simulink library "sm_wheel_loader_lib"  (R2025a)
settings: Solver=VariableStepAuto  StartTime=0.0  StopTime=10.0  RelTol=1e-3
undefined symbols (not defined in the file): AToTOrificeVector, BiPOrificeVector, boomHEArea, boomREArea, BToTOrificeVector, fluids, GRake, GToothL, GToothR, HMPST, HydFcnParams, logLoad, Position, PToAOrificeVector, PToBOrificeVector, RakeL, RakeR, testInput, Wheel_Loader, X, Y, Z
libraries: sm_lib x694, fl_lib x183, nesl_utility x74, SimscapeFluids_lib x62, sdl_lib x25, cvt_components_lib x25, simulink_extras x5, $bdroot x4, wheel_loader_contact_lib x4, ee_lib x2, SignalEditorBlockLib x1, batteryecm_lib x1
(part 10 of 26)

== system sm_wheel_loader_lib/Wheel Loader Vehicle/Actuators/Hydraulic/Actuator Steer ==
  Actuator Steer : SimscapeFluids_lib/Isothermal Liquid/Actuators/Double-Acting Actuator (IL)  single_fluid=true  mech_orientation=foundation.enum.MechOrientationTranslational.Positive  piston_area_A=HydFcnParams.steerActuator.headEndArea mm^2  piston_area_B=HydFcnParams.steerActuator.rodEndArea mm^2  stroke=HydFcnParams.steerActuator.stroke mm  dead_volume_A=1e-4 m^3  dead_volume_B=1e-4 m^3  pressure_spec=foundation.enum.pressure_spec.atmospheric  environment_pressure=0.101325 MPa  hardstop_model=simscape.enum.hardstop.smooth  stiff_coeff=1e8 N/m  damping_coeff=1e5 N/(m/s)  transition=0.1 mm  coeff_rest=0.7  v_tol=0.001 m/s  f_tol=0.001 N  cushion_A_spec=simscape.enum.onoff.off  area_plunger_A=boomHEArea/4 mm^2  length_plunger_A=5 mm  area_cushion_orifice_A=5 mm^2  area_leak_plunger_A=1e-7 m^2  p_crack_differential_A=0.01 MPa  press_max_differential_A=0.1 MPa  check_valve_area_max_A=1e-4 m^2  check_valve_area_leak_A=1e-10 m^2  smoothing_factor_A=0  cushion_B_spec=simscape.enum.onoff.off  area_plunger_B=boomREArea/4 mm^2  length_plunger_B=5 mm  area_cushion_orifice_B=5 mm^2  area_leak_plunger_B=1e-7 m^2  p_crack_differential_B=0.01 MPa  press_max_differential_B=0.1 MPa  check_valve_area_max_B=1e-4 m^2  check_valve_area_leak_B=1e-10 m^2  smoothing_factor_B=0  friction_spec=simscape.enum.onoff.on  breakaway_Coulomb_ratio=HydFcnParams.steerActuator.brkawyToCoulRatio  breakaway_velocity=HydFcnParams.steerActuator.brkawyVel m/s  preload_force=HydFcnParams.steerActuator.preloadForce N  Coulomb_coeff=HydFcnParams.steerActuator.coulForceCoef N/Pa  viscous_coeff=HydFcnParams.steerActuator.viscCoeff lbf/(in/s)  leakage_spec=simscape.enum.onoff.off  clearance=1e-4 m  piston_length=0.01 m  displacement_spec=foundation.enum.DisplacementSpec.Calculate  x0=testInput.Active.Steer.p(1)*1000 mm  dynamic_compressibility=simscape.enum.onoff.on  p0_A=HydFcnParams.steerActuator.initHEPr bar  p0_B=HydFcnParams.steerActuator.initREPr bar  p_nominal_A=0.101325 MPa  p_nominal_B=0.101325 MPa
      settings: InternalSimscapePortConfiguration="{\"Bottom\":[],\"Left\":[{\"id\":\"C\",\"label\":\"C\",\"type\":\"foundation.mechanical.translational.translational\"},{\"id\":\"A\",\"label\":\"A\",\"type\":\"foundation.isothermal_liquid.isothermal_liquid\"}],\"Right\":[{\"id\":\"p_out\",\"label\":\"p\",\"type\":\"output\"},{\"id\":\"R\",\"label\":\"R\",\"type\":\"foundation.mechanical.translational.translational\"},{\"id\":\"B\",\"label\":\"B\",\"type\":\"foundation.isothermal_liquid.isothermal_liquid\"}],\"Top\":[]}"
  MTRef : fl_lib/Mechanical/Translational Elements/Mechanical Translational Reference
  PS Terminator : fl_lib/Physical Signals/Sinks/PS Terminator
  A : PMIOPort  Side=Left
  B : PMIOPort  Port=2  Side=Left
  R : PMIOPort  Port=3  Side=Right
  connections:
  Actuator Steer/LConn1 -- MTRef/LConn1
  A/RConn1 -- Actuator Steer/LConn2
  B/RConn1 -- Actuator Steer/RConn3
  R/RConn1 -- Actuator Steer/RConn2
  Actuator Steer/RConn1 -- PS Terminator/LConn1

== system sm_wheel_loader_lib/Wheel Loader Vehicle/Actuators/Hydraulic/Controller ==
  note: Inputs - Outputs:
      |
      | Joystick position for lift (-1 to 1) velocity control - lift arm spool position
      | Joystick position for tilt (-1 to 1) velocity control - tilt spool position
  BusElementIn : Inport  PortName=Cmd  Element=LiftCmd
  BusElementIn1 : Inport  PortName=Cmd  Element=TiltCmd
  Gain : Gain  Gain=5
  Gain1 : Gain  Gain=5
  LiftSpoolPosCmdRateLimit : RateLimiter  RisingSlewLimit=HydFcnParams.liftActCtrl.posSpoolCmdRateLimit  FallingSlewLimit=HydFcnParams.liftActCtrl.negSpoolCmdRateLimit  SampleTimeMode=inherited
  LiftSpoolPosCmdSaturation : Saturate  UpperLimit=HydFcnParams.liftActCtrl.maxSpoolCmd  LowerLimit=HydFcnParams.liftActCtrl.minSpoolCmd
  TiltSpoolPosCmdRateLimit : RateLimiter  RisingSlewLimit=HydFcnParams.tiltActCtrl.posSpoolCmdRateLimit  FallingSlewLimit=HydFcnParams.tiltActCtrl.negSpoolCmdRateLimit  SampleTimeMode=inherited
  TiltSpoolPosCmdSaturation : Saturate  UpperLimit=HydFcnParams.tiltActCtrl.maxSpoolCmd  LowerLimit=HydFcnParams.tiltActCtrl.minSpoolCmd
  Out Bus Element : Outport  PortName=pSpool  Element=tilt
  Out Bus Element1 : Outport  PortName=pSpool  Element=lift
  wires:
  Gain/1 -> LiftSpoolPosCmdSaturation/1
  Gain1/1 -> TiltSpoolPosCmdSaturation/1
  LiftSpoolPosCmdSaturation/1 -> LiftSpoolPosCmdRateLimit/1
  TiltSpoolPosCmdSaturation/1 -> TiltSpoolPosCmdRateLimit/1
  LiftSpoolPosCmdRateLimit/1 -> Out Bus Element1/1  "LiftSpoolPosCmd"
  TiltSpoolPosCmdRateLimit/1 -> Out Bus Element/1  "TiltSpoolCmd"
  BusElementIn1/1 -> Gain1/1
  BusElementIn/1 -> Gain/1

== system sm_wheel_loader_lib/Wheel Loader Vehicle/Actuators/Hydraulic/Implement ==
  A : Inport
  Bucket : Subsystem  VariantControl=Bucket
      mask Display: image('sm_wheel_loader_actuator_bucket_IMAGE.png')
  Grapple : Subsystem  VariantControl=Grapple
      mask Display: image('sm_wheel_loader_actuator_grapple_IMAGE.png')
  Impl : PMIOPort  Side=Right

== system sm_wheel_loader_lib/Wheel Loader Vehicle/Actuators/Hydraulic/Valve Steer ==
  CV SteerA : SimscapeFluids_lib/Isothermal Liquid/Valves & Orifices/Directional Control Valves/Check Valve (IL)  opening_spec=2*(fluids.isothermal_liquid.valves_orifices.enum.opening_spec.linear)-1  pressure_control_spec=fluids.isothermal_liquid.valves_orifices.enum.pressure_control_spec.dp  p_crack_differential=HydFcnParams.checkValves.crackingPrDiff bar  p_crack_gauge=0.1 MPa  press_max_differential=HydFcnParams.checkValves.maxOpeningPrDiff bar  press_max_gauge=0.2 MPa  area_max=HydFcnParams.checkValves.maxOpeningArea mm^2  area_leak="HydFcnParams.checkValves.leakageArea  mm^2"  p_diff_TLU=[0.01 : 0.01 : 0.1] MPa  valve_area_TLU=[1e-10, 1e-05, 2e-05, 3e-05, 4e-05, 5e-05, 6e-05, 7.5e-05, 8.5e-05, .0001] m^2  vol_flow_TLU=[.000358, .045, .11, .191, .284, .39, .505, .63, .764, .905] .* 1e-3 m^3/s  area=inf m^2  Cd=HydFcnParams.checkValves.dischargeCoef  Re_c=HydFcnParams.checkValves.critReynoldsNmbr  smoothing_factor=HydFcnParams.checkValves.smoothingFactor  pressure_recovery=simscape.enum.onoff.off  opening_dynamics=simscape.enum.onoff.off  tau=0.1 s
      settings: InternalSimscapePortConfiguration="{\"Bottom\":[],\"Left\":[{\"id\":\"A\",\"label\":\"A\",\"type\":\"foundation.isothermal_liquid.isothermal_liquid\"}],\"Right\":[{\"id\":\"B\",\"label\":\"B\",\"type\":\"foundation.isothermal_liquid.isothermal_liquid\"}],\"Top\":[]}"
  CV SteerB : SimscapeFluids_lib/Isothermal Liquid/Valves & Orifices/Directional Control Valves/Check Valve (IL)  opening_spec=2*(fluids.isothermal_liquid.valves_orifices.enum.opening_spec.linear)-1  pressure_control_spec=fluids.isothermal_liquid.valves_orifices.enum.pressure_control_spec.dp  p_crack_differential=HydFcnParams.checkValves.crackingPrDiff bar  p_crack_gauge=0.1 MPa  press_max_differential=HydFcnParams.checkValves.maxOpeningPrDiff bar  press_max_gauge=0.2 MPa  area_max=HydFcnParams.checkValves.maxOpeningArea mm^2  area_leak="HydFcnParams.checkValves.leakageArea  mm^2"  p_diff_TLU=[0.01 : 0.01 : 0.1] MPa  valve_area_TLU=[1e-10, 1e-05, 2e-05, 3e-05, 4e-05, 5e-05, 6e-05, 7.5e-05, 8.5e-05, .0001] m^2  vol_flow_TLU=[.000358, .045, .11, .191, .284, .39, .505, .63, .764, .905] .* 1e-3 m^3/s  area=inf m^2  Cd=HydFcnParams.checkValves.dischargeCoef  Re_c=HydFcnParams.checkValves.critReynoldsNmbr  smoothing_factor=HydFcnParams.checkValves.smoothingFactor  pressure_recovery=simscape.enum.onoff.off  opening_dynamics=simscape.enum.onoff.off  tau=0.1 s
      settings: InternalSimscapePortConfiguration="{\"Bottom\":[],\"Left\":[{\"id\":\"A\",\"label\":\"A\",\"type\":\"foundation.isothermal_liquid.isothermal_liquid\"}],\"Right\":[{\"id\":\"B\",\"label\":\"B\",\"type\":\"foundation.isothermal_liquid.isothermal_liquid\"}],\"Top\":[]}"
  CV SteerP : SimscapeFluids_lib/Isothermal Liquid/Valves & Orifices/Directional Control Valves/Check Valve (IL)  opening_spec=2*(fluids.isothermal_liquid.valves_orifices.enum.opening_spec.linear)-1  pressure_control_spec=fluids.isothermal_liquid.valves_orifices.enum.pressure_control_spec.dp  p_crack_differential=HydFcnParams.checkValves.crackingPrDiff bar  p_crack_gauge=0.1 MPa  press_max_differential=HydFcnParams.checkValves.maxOpeningPrDiff bar  press_max_gauge=0.2 MPa  area_max=HydFcnParams.checkValves.maxOpeningArea mm^2  area_leak="HydFcnParams.checkValves.leakageArea  mm^2"  p_diff_TLU=[0.01 : 0.01 : 0.1] MPa  valve_area_TLU=[1e-10, 1e-05, 2e-05, 3e-05, 4e-05, 5e-05, 6e-05, 7.5e-05, 8.5e-05, .0001] m^2  vol_flow_TLU=[.000358, .045, .11, .191, .284, .39, .505, .63, .764, .905] .* 1e-3 m^3/s  area=inf m^2  Cd=HydFcnParams.checkValves.dischargeCoef  Re_c=HydFcnParams.checkValves.critReynoldsNmbr  smoothing_factor=HydFcnParams.checkValves.smoothingFactor  pressure_recovery=simscape.enum.onoff.off  opening_dynamics=simscape.enum.onoff.off  tau=0.1 s
      settings: InternalSimscapePortConfiguration="{\"Bottom\":[],\"Left\":[{\"id\":\"A\",\"label\":\"A\",\"type\":\"foundation.isothermal_liquid.isothermal_liquid\"}],\"Right\":[{\"id\":\"B\",\"label\":\"B\",\"type\":\"foundation.isothermal_liquid.isothermal_liquid\"}],\"Top\":[]}"
  CVC GerotorA : fl_lib/Isothermal Liquid/Elements/Constant Volume Chamber (IL)  volume=HydFcnParams.steerValve.gerChamberVol mm^3  p_I_specify=off  p_I_priority=High  p_I=0.101325 MPa  p_I_nominal_specify=off  p_I_nominal_value=1  p_I_nominal_unit=MPa
      settings: InternalSimscapePortConfiguration="{\"Bottom\":[],\"Left\":[{\"id\":\"A\",\"label\":\"A\",\"type\":\"foundation.isothermal_liquid.isothermal_liquid\"}],\"Right\":[],\"Top\":[]}"
  CVC GerotorB : fl_lib/Isothermal Liquid/Elements/Constant Volume Chamber (IL)  volume=HydFcnParams.steerValve.gerChamberVol mm^3  p_I_specify=off  p_I_priority=High  p_I=0.101325 MPa  p_I_nominal_specify=off  p_I_nominal_value=1  p_I_nominal_unit=MPa
      settings: InternalSimscapePortConfiguration="{\"Bottom\":[],\"Left\":[{\"id\":\"A\",\"label\":\"A\",\"type\":\"foundation.isothermal_liquid.isothermal_liquid\"}],\"Right\":[],\"Top\":[]}"
  CVC Steer A : fl_lib/Isothermal Liquid/Elements/Constant Volume Chamber (IL)  volume=HydFcnParams.steerValve.gerChamberVol mm^3  p_I_specify=off  p_I_priority=High  p_I=0.101325 MPa  p_I_nominal_specify=off  p_I_nominal_value=1  p_I_nominal_unit=MPa
      settings: InternalSimscapePortConfiguration="{\"Bottom\":[],\"Left\":[{\"id\":\"A\",\"label\":\"A\",\"type\":\"foundation.isothermal_liquid.isothermal_liquid\"}],\"Right\":[],\"Top\":[]}"
  CVC Steer B : fl_lib/Isothermal Liquid/Elements/Constant Volume Chamber (IL)  volume=HydFcnParams.steerValve.gerChamberVol mm^3  p_I_specify=off  p_I_priority=High  p_I=0.101325 MPa  p_I_nominal_specify=off  p_I_nominal_value=1  p_I_nominal_unit=MPa
      settings: InternalSimscapePortConfiguration="{\"Bottom\":[],\"Left\":[{\"id\":\"A\",\"label\":\"A\",\"type\":\"foundation.isothermal_liquid.isothermal_liquid\"}],\"Right\":[],\"Top\":[]}"
  Gerotor : SimscapeFluids_lib/Isothermal Liquid/Pumps & Motors/Fixed-Displacement Motor (IL)  leakage_friction_spec=fluids.isothermal_liquid.pumps_motors.enum.MotorLossSpec.InputEfficiency  displacement=HydFcnParams.steerValve.gerDisplacement cm^3/rev  omega_nominal=20 rpm  p_nominal=10 MPa  vol_eff_nominal=0.92  mech_eff_nominal=0.88  no_load_torque=0 N*m  p_diff_eff_TLU=[.1, 1, 2] MPa  omega_eff_TLU=[250, 500, 1000, 2000, 3000, 4000] rpm  vol_eff_TLU=[.816, .908, .954, .977, .981, .984; .325, .663, .831, .916, .925, .946; .137, .568, .78, .892, .893, .91]  mech_eff_TLU=[.996, .996, .996, .996, .996, .996; .988, .989, .989, .989, .989, .99; .981, .981, .982, .982, .983, .984]  p_diff_loss_TLU=[.1, 1, 2] MPa  omega_loss_TLU=[250, 500, 1000, 2000, 3000, 4000] rpm  vol_loss_TLU=1e-3 * [.023, .023, .023, .023, .0285, .032; .0844, .0842, .0845, .084, .1125, .108; .1079, .108, .11, .108, .1605, .18] m^3/s  mech_loss_TLU=[.002, .002, .002, .002, .002, .002; .0607, .0556, .0556, .0556, .0556, .0505; .1937, .1937, .1833, .1833, .1729, .1626] N*m  q_shaft_TLU=[.125, .25, .5, 1, 1.5, 2] * 1e-3 m^3/s  p_diff_shaft_TLU=[.1, 1, 2] MPa  torque_shaft_TLU=[.47, 4.72, 9.35; .47, 4.7, 9.36; .47, 4.7, 9.4; .47, 4.7, 9.41; .47, 4.7, 9.46; .47, 4.68, 9.5] N*m  omega_shaft_TLU=[205, 80, 35; 455, 330, 285; 955, 831, 780; 1950, 1830, 1780; 2940, 2775, 2680; 3940, 3780, 3640] rpm  vol_eff_min=1e-3  vol_eff_max=1  mech_eff_min=1e-3  mech_eff_max=1  pressure_threshold=1e-3 MPa  omega_threshold=100 rpm  supplied_range_check=simscape.enum.assert.action.none  motor_mode_check=simscape.enum.assert.action.none  pressure_check=simscape.enum.assert.action.none  p_min_valid=0.101325 MPa
      settings: InternalSimscapePortConfiguration="{\"Bottom\":[{\"id\":\"B\",\"label\":\"B\",\"type\":\"foundation.isothermal_liquid.isothermal_liquid\"}],\"Left\":[{\"id\":\"EV\",\"label\":\"EV\",\"type\":\"input\"},{\"id\":\"EM\",\"label\":\"EM\",\"type\":\"input\"}],\"Right\":[{\"id\":\"R\",\"label\":\"R\",\"type\":\"foundation.mechanical.rotational.rotational\"},{\"id\":\"C\",\"label\":\"C\",\"type\":\"foundation.mechanical.rotational.rotational\"}],\"Top\":[{\"id\":\"A\",\"label\":\"A\",\"type\":\"foundation.isothermal_liquid.isothermal_liquid\"}]}"
  MRRef Gerotor : fl_lib/Mechanical/Rotational Elements/Mechanical Rotational Reference
  Orifices : Subsystem
      mask Display: image('sm_wheel_loader_valve_steer_IMAGE.png');
  PRV Steer Pump : SimscapeFluids_lib/Isothermal Liquid/Valves & Orifices/Pressure Control Valves/Pressure Relief Valve (IL)  set_pressure_spec=foundation.enum.constant_controlled.constant  opening_spec=fluids.isothermal_liquid.valves_orifices.enum.opening_spec.linear  pressure_spec=fluids.isothermal_liquid.valves_orifices.enum.pressure_control_spec.dp  p_set_gauge=0.1 MPa  p_set_differential=HydFcnParams.pumpPRV.reliefPr bar  p_range=HydFcnParams.pumpPRV.regRange bar  area_max=HydFcnParams.pumpPRV.maxOpeningArea mm^2  area_leak=HydFcnParams.pumpPRV.leakageArea mm^2  p_diff_TLU=[30.15e5 : 15e3 : 31.35e5] Pa  p_gauge_TLU=[30.15e5 : 15e3 : 31.35e5] Pa  valve_area_TLU=[1 : 1 : 9] .* 1e-5 m^2  vol_flow_TLU=[1e-09, 3.6e-05, 8.9e-05, .00015, .00023, .00031] m^3/s  area=inf m^2  Cd=HydFcnParams.pumpPRV.dischargeCoef  Re_c=HydFcnParams.pumpPRV.critReynoldsNmbr  smoothing_factor=HydFcnParams.pumpPRV.smoothingFactor  pressure_recovery=simscape.enum.onoff.off  opening_dynamics=simscape.enum.onoff.off  tau=0.1 s
      settings: InternalSimscapePortConfiguration="{\"Bottom\":[],\"Left\":[{\"id\":\"A\",\"label\":\"A\",\"type\":\"foundation.isothermal_liquid.isothermal_liquid\"}],\"Right\":[{\"id\":\"B\",\"label\":\"B\",\"type\":\"foundation.isothermal_liquid.isothermal_liquid\"}],\"Top\":[]}"
  PRV SteerA : SimscapeFluids_lib/Isothermal Liquid/Valves & Orifices/Pressure Control Valves/Pressure Relief Valve (IL)  set_pressure_spec=foundation.enum.constant_controlled.constant  opening_spec=fluids.isothermal_liquid.valves_orifices.enum.opening_spec.linear  pressure_spec=fluids.isothermal_liquid.valves_orifices.enum.pressure_control_spec.dp  p_set_gauge=0.1 MPa  p_set_differential=HydFcnParams.actPRV.reliefPr bar  p_range=HydFcnParams.actPRV.regRange bar  area_max=HydFcnParams.actPRV.maxOpeningArea mm^2  area_leak=HydFcnParams.actPRV.leakageArea mm^2  p_diff_TLU=[30.15e5 : 15e3 : 31.35e5] Pa  p_gauge_TLU=[30.15e5 : 15e3 : 31.35e5] Pa  valve_area_TLU=[1 : 1 : 9] .* 1e-5 m^2  vol_flow_TLU=[1e-09, 3.6e-05, 8.9e-05, .00015, .00023, .00031] m^3/s  area=inf m^2  Cd=HydFcnParams.actPRV.dischargeCoef  Re_c=HydFcnParams.actPRV.critReynoldsNmbr  smoothing_factor=HydFcnParams.actPRV.smoothingFactor  pressure_recovery=simscape.enum.onoff.off  opening_dynamics=simscape.enum.onoff.off  tau=0.1 s
      settings: InternalSimscapePortConfiguration="{\"Bottom\":[],\"Left\":[{\"id\":\"A\",\"label\":\"A\",\"type\":\"foundation.isothermal_liquid.isothermal_liquid\"}],\"Right\":[{\"id\":\"B\",\"label\":\"B\",\"type\":\"foundation.isothermal_liquid.isothermal_liquid\"}],\"Top\":[]}"
  PRV SteerB : SimscapeFluids_lib/Isothermal Liquid/Valves & Orifices/Pressure Control Valves/Pressure Relief Valve (IL)  set_pressure_spec=foundation.enum.constant_controlled.constant  opening_spec=fluids.isothermal_liquid.valves_orifices.enum.opening_spec.linear  pressure_spec=fluids.isothermal_liquid.valves_orifices.enum.pressure_control_spec.dp  p_set_gauge=0.1 MPa  p_set_differential=HydFcnParams.actPRV.reliefPr bar  p_range=HydFcnParams.actPRV.regRange bar  area_max=HydFcnParams.actPRV.maxOpeningArea mm^2  area_leak=HydFcnParams.actPRV.leakageArea mm^2  p_diff_TLU=[30.15e5 : 15e3 : 31.35e5] Pa  p_gauge_TLU=[30.15e5 : 15e3 : 31.35e5] Pa  valve_area_TLU=[1 : 1 : 9] .* 1e-5 m^2  vol_flow_TLU=[1e-09, 3.6e-05, 8.9e-05, .00015, .00023, .00031] m^3/s  area=inf m^2  Cd=HydFcnParams.actPRV.dischargeCoef  Re_c=HydFcnParams.actPRV.critReynoldsNmbr  smoothing_factor=HydFcnParams.actPRV.smoothingFactor  pressure_recovery=simscape.enum.onoff.off  opening_dynamics=simscape.enum.onoff.off  tau=0.1 s
      settings: InternalSimscapePortConfiguration="{\"Bottom\":[],\"Left\":[{\"id\":\"A\",\"label\":\"A\",\"type\":\"foundation.isothermal_liquid.isothermal_liquid\"}],\"Right\":[{\"id\":\"B\",\"label\":\"B\",\"type\":\"foundation.isothermal_liquid.isothermal_liquid\"}],\"Top\":[]}"
  PS Constant : fl_lib/Physical Signals/Sources/PS Constant  constant=1
  Sleeve Damper : fl_lib/Mechanical/Rotational Elements/Rotational Damper  D=HydFcnParams.steerValve.sleeveDamping N*m*s/rad  w_specify=off  w_priority=None  w=0 rad/s  w_nominal_specify=off  w_nominal_value=1  w_nominal_unit=rad/s  t_specify=off  t_priority=None  t=0 N*m  t_nominal_specify=off  t_nominal_value=1  t_nominal_unit=N*m
  Sleeve Deflection : fl_lib/Mechanical/Mechanical Sensors/Ideal Rotational Motion Sensor  reference=foundation.enum.MeasurementReference.difference  acceleration_port=false  velocity_port=false  position_port=true  wrap_angle=false  offset=0 rad
      settings: InternalSimscapePortConfiguration="{\"Bottom\":[],\"Left\":[{\"id\":\"R\",\"label\":\"R\",\"type\":\"foundation.mechanical.rotational.rotational\"}],\"Right\":[{\"id\":\"C\",\"label\":\"C\",\"type\":\"foundation.mechanical.rotational.rotational\"},{\"id\":\"A\",\"label\":\"A\",\"type\":\"output\"}],\"Top\":[]}"
  Sleeve Hard Stop : fl_lib/Mechanical/Rotational Elements/Rotational Hard Stop  upper_bnd=HydFcnParams.steerValve.maxRelAngle rad  lower_bnd=HydFcnParams.steerValve.minRelAngle rad  model=simscape.enum.hardstop.smooth  stiff_up=HydFcnParams.steerValve.hardstopStiff N*m/rad  stiff_low=HydFcnParams.steerValve.hardstopStiff N*m/rad  D_up=HydFcnParams.steerValve.hardstopDamping N*m*s/rad  D_low=HydFcnParams.steerValve.hardstopDamping N*m*s/rad  transition=0.0001 rad  coeff_rest=0.7  w_tol=0.1 rad/s  trq_tol=0.001 N*m  w_specify=off  w_priority=None  w=0 rad/s  w_nominal_specify=off  w_nominal_value=1  w_nominal_unit=rad/s  t_specify=off  t_priority=None  t=0 N*m  t_nominal_specify=off  t_nominal_value=1  t_nominal_unit=N*m  phi_specify=off  phi_priority=High  phi=0 rad  phi_nominal_specify=off  phi_nominal_value=1  phi_nominal_unit=rad  M_specify=off  M_priority=None  M=0
  Sleeve Inertia : fl_lib/Mechanical/Rotational Elements/Inertia  inertia=0.01*10 kg*m^2  num_ports=foundation.enum.numPorts2.two  w_specify=off  w_priority=High  w=0 rad/s  w_nominal_specify=off  w_nominal_value=1  w_nominal_unit=rad/s  t_specify=off  t_priority=None  t=0 N*m  t_nominal_specify=off  t_nominal_value=1  t_nominal_unit=N*m
      settings: InternalSimscapePortConfiguration="{\"Bottom\":[],\"Left\":[{\"id\":\"I\",\"label\":\"\",\"type\":\"foundation.mechanical.rotational.rotational\"}],\"Right\":[{\"id\":\"J\",\"label\":\"\",\"type\":\"foundation.mechanical.rotational.rotational\"}],\"Top\":[]}"
  Sleeve Spring : fl_lib/Mechanical/Rotational Elements/Rotational Spring  spr_rate=HydFcnParams.steerValve.sleeveSpringStiff N*m/rad  w_specify=off  w_priority=None  w=0 rad/s  w_nominal_specify=off  w_nominal_value=1  w_nominal_unit=rad/s  t_specify=off  t_priority=None  t=0 N*m  t_nominal_specify=off  t_nominal_value=1  t_nominal_unit=N*m  phi_specify=off  phi_priority=High  phi=0 rad  phi_nominal_specify=off  phi_nominal_value=1  phi_nominal_unit=rad
  qSleeve to xSpool : Subsystem
  P : PMIOPort  Side=Left
  T : PMIOPort  Port=2  Side=Left
  A : PMIOPort  Port=3  Side=Right
  B : PMIOPort  Port=4  Side=Right
  SW : PMIOPort  Port=5  Side=Left
  connections:
  CV SteerB/RConn1 -- PRV SteerB/LConn1 -- Orifices/RConn4 -- B/RConn1 -- CVC Steer B/LConn1
  A/RConn1 -- CVC Steer A/LConn1 -- PRV SteerA/LConn1 -- CV SteerA/RConn1 -- Orifices/RConn1
  P/RConn1 -- CV SteerP/LConn1 -- PRV Steer Pump/LConn1
  PRV SteerA/RConn1 -- CV SteerA/LConn1 -- Orifices/LConn3 -- T/RConn1 -- PRV Steer Pump/RConn1 -- PRV SteerB/RConn1 -- CV SteerB/LConn1
  CV SteerP/RConn1 -- Orifices/LConn2
  Orifices/LConn1 -- qSleeve to xSpool/RConn1
  PS Constant/RConn1 -- Gerotor/LConn2 -- Gerotor/LConn1
  Gerotor/RConn3 -- Orifices/RConn3 -- CVC GerotorB/LConn1
  MRRef Gerotor/LConn1 -- Gerotor/RConn2
  Sleeve Inertia/RConn1 -- Gerotor/RConn1
  Gerotor/LConn3 -- CVC GerotorA/LConn1 -- Orifices/RConn2
  Sleeve Spring/RConn1 -- Sleeve Deflection/RConn1 -- Sleeve Hard Stop/RConn1 -- Sleeve Damper/RConn1 -- SW/RConn1
  Sleeve Hard Stop/LConn1 -- Sleeve Deflection/LConn1 -- Sleeve Inertia/LConn1 -- Sleeve Spring/LConn1 -- Sleeve Damper/LConn1
  qSleeve to xSpool/LConn1 -- Sleeve Deflection/RConn2

== system sm_wheel_loader_lib/Wheel Loader Vehicle/Actuators/Hydraulic/Valves Linkage ==
  In Bus Element : Inport  PortName=S  Element=tilt
  In Bus Element1 : Inport  PortName=S  Element=lift
  CV LiftA : SimscapeFluids_lib/Isothermal Liquid/Valves & Orifices/Directional Control Valves/Check Valve (IL)  opening_spec=2*(fluids.isothermal_liquid.valves_orifices.enum.opening_spec.linear)-1  pressure_control_spec=fluids.isothermal_liquid.valves_orifices.enum.pressure_control_spec.dp  p_crack_differential=HydFcnParams.checkValves.crackingPrDiff bar  p_crack_gauge=0.1 MPa  press_max_differential=HydFcnParams.checkValves.maxOpeningPrDiff bar  press_max_gauge=0.2 MPa  area_max=HydFcnParams.checkValves.maxOpeningArea mm^2  area_leak="HydFcnParams.checkValves.leakageArea  mm^2"  p_diff_TLU=[0.01 : 0.01 : 0.1] MPa  valve_area_TLU=[1e-10, 1e-05, 2e-05, 3e-05, 4e-05, 5e-05, 6e-05, 7.5e-05, 8.5e-05, .0001] m^2  vol_flow_TLU=[.000358, .045, .11, .191, .284, .39, .505, .63, .764, .905] .* 1e-3 m^3/s  area=inf m^2  Cd=HydFcnParams.checkValves.dischargeCoef  Re_c=HydFcnParams.checkValves.critReynoldsNmbr  smoothing_factor=HydFcnParams.checkValves.smoothingFactor  pressure_recovery=simscape.enum.onoff.off  opening_dynamics=simscape.enum.onoff.off  tau=0.1 s
      settings: InternalSimscapePortConfiguration="{\"Bottom\":[],\"Left\":[{\"id\":\"A\",\"label\":\"A\",\"type\":\"foundation.isothermal_liquid.isothermal_liquid\"}],\"Right\":[{\"id\":\"B\",\"label\":\"B\",\"type\":\"foundation.isothermal_liquid.isothermal_liquid\"}],\"Top\":[]}"
  CV LiftB : SimscapeFluids_lib/Isothermal Liquid/Valves & Orifices/Directional Control Valves/Check Valve (IL)  opening_spec=2*(fluids.isothermal_liquid.valves_orifices.enum.opening_spec.linear)-1  pressure_control_spec=fluids.isothermal_liquid.valves_orifices.enum.pressure_control_spec.dp  p_crack_differential=HydFcnParams.checkValves.crackingPrDiff bar  p_crack_gauge=0.1 MPa  press_max_differential=HydFcnParams.checkValves.maxOpeningPrDiff bar  press_max_gauge=0.2 MPa  area_max=HydFcnParams.checkValves.maxOpeningArea mm^2  area_leak="HydFcnParams.checkValves.leakageArea  mm^2"  p_diff_TLU=[0.01 : 0.01 : 0.1] MPa  valve_area_TLU=[1e-10, 1e-05, 2e-05, 3e-05, 4e-05, 5e-05, 6e-05, 7.5e-05, 8.5e-05, .0001] m^2  vol_flow_TLU=[.000358, .045, .11, .191, .284, .39, .505, .63, .764, .905] .* 1e-3 m^3/s  area=inf m^2  Cd=HydFcnParams.checkValves.dischargeCoef  Re_c=HydFcnParams.checkValves.critReynoldsNmbr  smoothing_factor=HydFcnParams.checkValves.smoothingFactor  pressure_recovery=simscape.enum.onoff.off  opening_dynamics=simscape.enum.onoff.off  tau=0.1 s
      settings: InternalSimscapePortConfiguration="{\"Bottom\":[],\"Left\":[{\"id\":\"A\",\"label\":\"A\",\"type\":\"foundation.isothermal_liquid.isothermal_liquid\"}],\"Right\":[{\"id\":\"B\",\"label\":\"B\",\"type\":\"foundation.isothermal_liquid.isothermal_liquid\"}],\"Top\":[]}"
  CV TiltA : SimscapeFluids_lib/Isothermal Liquid/Valves & Orifices/Directional Control Valves/Check Valve (IL)  opening_spec=2*(fluids.isothermal_liquid.valves_orifices.enum.opening_spec.linear)-1  pressure_control_spec=fluids.isothermal_liquid.valves_orifices.enum.pressure_control_spec.dp  p_crack_differential=HydFcnParams.checkValves.crackingPrDiff bar  p_crack_gauge=0.1 MPa  press_max_differential=HydFcnParams.checkValves.maxOpeningPrDiff bar  press_max_gauge=0.2 MPa  area_max=HydFcnParams.checkValves.maxOpeningArea mm^2  area_leak="HydFcnParams.checkValves.leakageArea  mm^2"  p_diff_TLU=[0.01 : 0.01 : 0.1] MPa  valve_area_TLU=[1e-10, 1e-05, 2e-05, 3e-05, 4e-05, 5e-05, 6e-05, 7.5e-05, 8.5e-05, .0001] m^2  vol_flow_TLU=[.000358, .045, .11, .191, .284, .39, .505, .63, .764, .905] .* 1e-3 m^3/s  area=inf m^2  Cd=HydFcnParams.checkValves.dischargeCoef  Re_c=HydFcnParams.checkValves.critReynoldsNmbr  smoothing_factor=HydFcnParams.checkValves.smoothingFactor  pressure_recovery=simscape.enum.onoff.off  opening_dynamics=simscape.enum.onoff.off  tau=0.1 s
      settings: InternalSimscapePortConfiguration="{\"Bottom\":[],\"Left\":[{\"id\":\"A\",\"label\":\"A\",\"type\":\"foundation.isothermal_liquid.isothermal_liquid\"}],\"Right\":[{\"id\":\"B\",\"label\":\"B\",\"type\":\"foundation.isothermal_liquid.isothermal_liquid\"}],\"Top\":[]}"
  CV TiltB : SimscapeFluids_lib/Isothermal Liquid/Valves & Orifices/Directional Control Valves/Check Valve (IL)  opening_spec=2*(fluids.isothermal_liquid.valves_orifices.enum.opening_spec.linear)-1  pressure_control_spec=fluids.isothermal_liquid.valves_orifices.enum.pressure_control_spec.dp  p_crack_differential=HydFcnParams.checkValves.crackingPrDiff bar  p_crack_gauge=0.1 MPa  press_max_differential=HydFcnParams.checkValves.maxOpeningPrDiff bar  press_max_gauge=0.2 MPa  area_max=HydFcnParams.checkValves.maxOpeningArea mm^2  area_leak="HydFcnParams.checkValves.leakageArea  mm^2"  p_diff_TLU=[0.01 : 0.01 : 0.1] MPa  valve_area_TLU=[1e-10, 1e-05, 2e-05, 3e-05, 4e-05, 5e-05, 6e-05, 7.5e-05, 8.5e-05, .0001] m^2  vol_flow_TLU=[.000358, .045, .11, .191, .284, .39, .505, .63, .764, .905] .* 1e-3 m^3/s  area=inf m^2  Cd=HydFcnParams.checkValves.dischargeCoef  Re_c=HydFcnParams.checkValves.critReynoldsNmbr  smoothing_factor=HydFcnParams.checkValves.smoothingFactor  pressure_recovery=simscape.enum.onoff.off  opening_dynamics=simscape.enum.onoff.off  tau=0.1 s
      settings: InternalSimscapePortConfiguration="{\"Bottom\":[],\"Left\":[{\"id\":\"A\",\"label\":\"A\",\"type\":\"foundation.isothermal_liquid.isothermal_liquid\"}],\"Right\":[{\"id\":\"B\",\"label\":\"B\",\"type\":\"foundation.isothermal_liquid.isothermal_liquid\"}],\"Top\":[]}"
  CV Lift : SimscapeFluids_lib/Isothermal Liquid/Valves & Orifices/Directional Control Valves/Check Valve (IL)  opening_spec=2*(fluids.isothermal_liquid.valves_orifices.enum.opening_spec.linear)-1  pressure_control_spec=fluids.isothermal_liquid.valves_orifices.enum.pressure_control_spec.dp  p_crack_differential=HydFcnParams.checkValves.crackingPrDiff bar  p_crack_gauge=0.1 MPa  press_max_differential=HydFcnParams.checkValves.maxOpeningPrDiff bar  press_max_gauge=0.2 MPa  area_max=HydFcnParams.checkValves.maxOpeningArea mm^2  area_leak="HydFcnParams.checkValves.leakageArea  mm^2"  p_diff_TLU=[0.01 : 0.01 : 0.1] MPa  valve_area_TLU=[1e-10, 1e-05, 2e-05, 3e-05, 4e-05, 5e-05, 6e-05, 7.5e-05, 8.5e-05, .0001] m^2  vol_flow_TLU=[.000358, .045, .11, .191, .284, .39, .505, .63, .764, .905] .* 1e-3 m^3/s  area=inf m^2  Cd=HydFcnParams.checkValves.dischargeCoef  Re_c=HydFcnParams.checkValves.critReynoldsNmbr  smoothing_factor=HydFcnParams.checkValves.smoothingFactor  pressure_recovery=simscape.enum.onoff.off  opening_dynamics=simscape.enum.onoff.off  tau=0.1 s
      settings: InternalSimscapePortConfiguration="{\"Bottom\":[],\"Left\":[{\"id\":\"A\",\"label\":\"A\",\"type\":\"foundation.isothermal_liquid.isothermal_liquid\"}],\"Right\":[{\"id\":\"B\",\"label\":\"B\",\"type\":\"foundation.isothermal_liquid.isothermal_liquid\"}],\"Top\":[]}"
  CV Tilt : SimscapeFluids_lib/Isothermal Liquid/Valves & Orifices/Directional Control Valves/Check Valve (IL)  opening_spec=2*(fluids.isothermal_liquid.valves_orifices.enum.opening_spec.linear)-1  pressure_control_spec=fluids.isothermal_liquid.valves_orifices.enum.pressure_control_spec.dp  p_crack_differential=HydFcnParams.checkValves.crackingPrDiff bar  p_crack_gauge=0.1 MPa  press_max_differential=HydFcnParams.checkValves.maxOpeningPrDiff bar  press_max_gauge=0.2 MPa  area_max=HydFcnParams.checkValves.maxOpeningArea mm^2  area_leak="HydFcnParams.checkValves.leakageArea  mm^2"  p_diff_TLU=[0.01 : 0.01 : 0.1] MPa  valve_area_TLU=[1e-10, 1e-05, 2e-05, 3e-05, 4e-05, 5e-05, 6e-05, 7.5e-05, 8.5e-05, .0001] m^2  vol_flow_TLU=[.000358, .045, .11, .191, .284, .39, .505, .63, .764, .905] .* 1e-3 m^3/s  area=inf m^2  Cd=HydFcnParams.checkValves.dischargeCoef  Re_c=HydFcnParams.checkValves.critReynoldsNmbr  smoothing_factor=HydFcnParams.checkValves.smoothingFactor  pressure_recovery=simscape.enum.onoff.off  opening_dynamics=simscape.enum.onoff.off  tau=0.1 s
      settings: InternalSimscapePortConfiguration="{\"Bottom\":[],\"Left\":[{\"id\":\"A\",\"label\":\"A\",\"type\":\"foundation.isothermal_liquid.isothermal_liquid\"}],\"Right\":[{\"id\":\"B\",\"label\":\"B\",\"type\":\"foundation.isothermal_liquid.isothermal_liquid\"}],\"Top\":[]}"
  Flow Divider : Subsystem
      mask Display: image('sm_wheel_loader_flow_divider_IMAGE.png');
  Orifices Lift : Subsystem  mask{valveData=HydFcnParams.liftValve}
      mask prompts: valveData "Lift Valve Data Structure:"
      mask DialogControl DescGroupVar Prompt: Lift Valve
      mask DialogControl DescTextVar Prompt: The Lift Valve is an open center 6/3 directional control valve
      mask Display: image('sm_wheel_loader_valve_lift_IMAGE.png')
  Orifices Tilt : Subsystem  mask{valveData=HydFcnParams.tiltValve}
      mask prompts: valveData "Tilt Valve Data Structure:"
      mask DialogControl DescGroupVar Prompt: Tilt Valve
      mask DialogControl DescTextVar Prompt: The Tilt Valve is an open center 6/3 directional control valve
      mask Display: image('sm_wheel_loader_valve_tilt_IMAGE.png');
  PRV LiftA : SimscapeFluids_lib/Isothermal Liquid/Valves & Orifices/Pressure Control Valves/Pressure Relief Valve (IL)  set_pressure_spec=foundation.enum.constant_controlled.constant  opening_spec=fluids.isothermal_liquid.valves_orifices.enum.opening_spec.linear  pressure_spec=fluids.isothermal_liquid.valves_orifices.enum.pressure_control_spec.dp  p_set_gauge=0.1 MPa  p_set_differential=HydFcnParams.actPRV.reliefPr bar  p_range=HydFcnParams.actPRV.regRange bar  area_max=HydFcnParams.actPRV.maxOpeningArea mm^2  area_leak=HydFcnParams.actPRV.leakageArea mm^2  p_diff_TLU=[30.15e5 : 15e3 : 31.35e5] Pa  p_gauge_TLU=[30.15e5 : 15e3 : 31.35e5] Pa  valve_area_TLU=[1 : 1 : 9] .* 1e-5 m^2  vol_flow_TLU=[1e-09, 3.6e-05, 8.9e-05, .00015, .00023, .00031] m^3/s  area=inf m^2  Cd=HydFcnParams.actPRV.dischargeCoef  Re_c=HydFcnParams.actPRV.critReynoldsNmbr  smoothing_factor=HydFcnParams.actPRV.smoothingFactor  pressure_recovery=simscape.enum.onoff.off  opening_dynamics=simscape.enum.onoff.off  tau=0.1 s
      settings: InternalSimscapePortConfiguration="{\"Bottom\":[],\"Left\":[{\"id\":\"A\",\"label\":\"A\",\"type\":\"foundation.isothermal_liquid.isothermal_liquid\"}],\"Right\":[{\"id\":\"B\",\"label\":\"B\",\"type\":\"foundation.isothermal_liquid.isothermal_liquid\"}],\"Top\":[]}"
  PRV LiftB : SimscapeFluids_lib/Isothermal Liquid/Valves & Orifices/Pressure Control Valves/Pressure Relief Valve (IL)  set_pressure_spec=foundation.enum.constant_controlled.constant  opening_spec=fluids.isothermal_liquid.valves_orifices.enum.opening_spec.linear  pressure_spec=fluids.isothermal_liquid.valves_orifices.enum.pressure_control_spec.dp  p_set_gauge=0.1 MPa  p_set_differential=HydFcnParams.actPRV.reliefPr bar  p_range=HydFcnParams.actPRV.regRange bar  area_max=HydFcnParams.actPRV.maxOpeningArea mm^2  area_leak=HydFcnParams.actPRV.leakageArea mm^2  p_diff_TLU=[30.15e5 : 15e3 : 31.35e5] Pa  p_gauge_TLU=[30.15e5 : 15e3 : 31.35e5] Pa  valve_area_TLU=[1 : 1 : 9] .* 1e-5 m^2  vol_flow_TLU=[1e-09, 3.6e-05, 8.9e-05, .00015, .00023, .00031] m^3/s  area=inf m^2  Cd=HydFcnParams.actPRV.dischargeCoef  Re_c=HydFcnParams.actPRV.critReynoldsNmbr  smoothing_factor=HydFcnParams.actPRV.smoothingFactor  pressure_recovery=simscape.enum.onoff.off  opening_dynamics=simscape.enum.onoff.off  tau=0.1 s
      settings: InternalSimscapePortConfiguration="{\"Bottom\":[],\"Left\":[{\"id\":\"A\",\"label\":\"A\",\"type\":\"foundation.isothermal_liquid.isothermal_liquid\"}],\"Right\":[{\"id\":\"B\",\"label\":\"B\",\"type\":\"foundation.isothermal_liquid.isothermal_liquid\"}],\"Top\":[]}"
  PRV Pump : SimscapeFluids_lib/Isothermal Liquid/Valves & Orifices/Pressure Control Valves/Pressure Relief Valve (IL)  set_pressure_spec=foundation.enum.constant_controlled.constant  opening_spec=fluids.isothermal_liquid.valves_orifices.enum.opening_spec.linear  pressure_spec=fluids.isothermal_liquid.valves_orifices.enum.pressure_control_spec.dp  p_set_gauge=0.1 MPa  p_set_differential=HydFcnParams.pumpPRV.reliefPr bar  p_range=HydFcnParams.pumpPRV.regRange bar  area_max=HydFcnParams.pumpPRV.maxOpeningArea mm^2  area_leak=HydFcnParams.pumpPRV.leakageArea mm^2  p_diff_TLU=[30.15e5 : 15e3 : 31.35e5] Pa  p_gauge_TLU=[30.15e5 : 15e3 : 31.35e5] Pa  valve_area_TLU=[1 : 1 : 9] .* 1e-5 m^2  vol_flow_TLU=[1e-09, 3.6e-05, 8.9e-05, .00015, .00023, .00031] m^3/s  area=inf m^2  Cd=HydFcnParams.pumpPRV.dischargeCoef  Re_c=HydFcnParams.pumpPRV.critReynoldsNmbr  smoothing_factor=HydFcnParams.pumpPRV.smoothingFactor  pressure_recovery=simscape.enum.onoff.off  opening_dynamics=simscape.enum.onoff.off  tau=0.1 s
      settings: InternalSimscapePortConfiguration="{\"Bottom\":[],\"Left\":[{\"id\":\"A\",\"label\":\"A\",\"type\":\"foundation.isothermal_liquid.isothermal_liquid\"}],\"Right\":[{\"id\":\"B\",\"label\":\"B\",\"type\":\"foundation.isothermal_liquid.isothermal_liquid\"}],\"Top\":[]}"
  PRV TiltA : SimscapeFluids_lib/Isothermal Liquid/Valves & Orifices/Pressure Control Valves/Pressure Relief Valve (IL)  set_pressure_spec=foundation.enum.constant_controlled.constant  opening_spec=fluids.isothermal_liquid.valves_orifices.enum.opening_spec.linear  pressure_spec=fluids.isothermal_liquid.valves_orifices.enum.pressure_control_spec.dp  p_set_gauge=0.1 MPa  p_set_differential=HydFcnParams.actPRV.reliefPr bar  p_range=HydFcnParams.actPRV.regRange bar  area_max=HydFcnParams.actPRV.maxOpeningArea mm^2  area_leak=HydFcnParams.actPRV.leakageArea mm^2  p_diff_TLU=[30.15e5 : 15e3 : 31.35e5] Pa  p_gauge_TLU=[30.15e5 : 15e3 : 31.35e5] Pa  valve_area_TLU=[1 : 1 : 9] .* 1e-5 m^2  vol_flow_TLU=[1e-09, 3.6e-05, 8.9e-05, .00015, .00023, .00031] m^3/s  area=inf m^2  Cd=HydFcnParams.actPRV.dischargeCoef  Re_c=HydFcnParams.actPRV.critReynoldsNmbr  smoothing_factor=HydFcnParams.actPRV.smoothingFactor  pressure_recovery=simscape.enum.onoff.off  opening_dynamics=simscape.enum.onoff.off  tau=0.1 s
      settings: InternalSimscapePortConfiguration="{\"Bottom\":[],\"Left\":[{\"id\":\"A\",\"label\":\"A\",\"type\":\"foundation.isothermal_liquid.isothermal_liquid\"}],\"Right\":[{\"id\":\"B\",\"label\":\"B\",\"type\":\"foundation.isothermal_liquid.isothermal_liquid\"}],\"Top\":[]}"
  PRV TiltB : SimscapeFluids_lib/Isothermal Liquid/Valves & Orifices/Pressure Control Valves/Pressure Relief Valve (IL)  set_pressure_spec=foundation.enum.constant_controlled.constant  opening_spec=fluids.isothermal_liquid.valves_orifices.enum.opening_spec.linear  pressure_spec=fluids.isothermal_liquid.valves_orifices.enum.pressure_control_spec.dp  p_set_gauge=0.1 MPa  p_set_differential=HydFcnParams.actPRV.reliefPr bar  p_range=HydFcnParams.actPRV.regRange bar  area_max=HydFcnParams.actPRV.maxOpeningArea mm^2  area_leak=HydFcnParams.actPRV.leakageArea mm^2  p_diff_TLU=[30.15e5 : 15e3 : 31.35e5] Pa  p_gauge_TLU=[30.15e5 : 15e3 : 31.35e5] Pa  valve_area_TLU=[1 : 1 : 9] .* 1e-5 m^2  vol_flow_TLU=[1e-09, 3.6e-05, 8.9e-05, .00015, .00023, .00031] m^3/s  area=inf m^2  Cd=HydFcnParams.actPRV.dischargeCoef  Re_c=HydFcnParams.actPRV.critReynoldsNmbr  smoothing_factor=HydFcnParams.actPRV.smoothingFactor  pressure_recovery=simscape.enum.onoff.off  opening_dynamics=simscape.enum.onoff.off  tau=0.1 s
      settings: InternalSimscapePortConfiguration="{\"Bottom\":[],\"Left\":[{\"id\":\"A\",\"label\":\"A\",\"type\":\"foundation.isothermal_liquid.isothermal_liquid\"}],\"Right\":[{\"id\":\"B\",\"label\":\"B\",\"type\":\"foundation.isothermal_liquid.isothermal_liquid\"}],\"Top\":[]}"
  Simulink-PS Converter : nesl_utility/Simulink-PS Converter  PhysicalDomain=network_engine_domain  SubClassName=ps_input  LeftPortType=input  RightPortType=output  PseudoPeriodic=off  Frequencies=[]  NoiseDistribution=none  NoiseParameters=[]  Unit=mm  AffineConversion=off  FilteringAndDerivatives=provide  SimscapeFilterOrder=1  InputFilterTimeConstant=0.001  UdotUserProvided=0
  Simulink-PS Converter1 : nesl_utility/Simulink-PS Converter  PhysicalDomain=network_engine_domain  SubClassName=ps_input  LeftPortType=input  RightPortType=output  PseudoPeriodic=off  Frequencies=[]  NoiseDistribution=none  NoiseParameters=[]  Unit=mm  AffineConversion=off  FilteringAndDerivatives=provide  SimscapeFilterOrder=1  InputFilterTimeConstant=0.001  UdotUserProvided=0
  P : PMIOPort  Side=Left
  T : PMIOPort  Port=2  Side=Left
  LiftA : PMIOPort  Port=3  Side=Right
  LiftB : PMIOPort  Port=4  Side=Right
  TiltA : PMIOPort  Port=5  Side=Right
  TiltB : PMIOPort  Port=6  Side=Right
  wires:
  In Bus Element/1 -> Simulink-PS Converter/1
  In Bus Element1/1 -> Simulink-PS Converter1/1
  connections:
  LiftB/RConn1 -- Orifices Lift/RConn2 -- CV LiftA/RConn1 -- PRV LiftB/LConn1
  LiftA/RConn1 -- Orifices Lift/RConn1 -- CV LiftB/RConn1 -- PRV LiftA/LConn1
  Orifices Lift/LConn4 -- CV Lift/RConn1 -- Orifices Lift/LConn2
  Orifices Tilt/RConn2 -- CV TiltB/RConn1 -- PRV TiltB/LConn1 -- TiltB/RConn1
  Orifices Tilt/RConn1 -- TiltA/RConn1 -- CV TiltA/RConn1 -- PRV TiltA/LConn1
  Orifices Tilt/LConn4 -- CV Tilt/RConn1 -- Orifices Tilt/LConn2
  Orifices Lift/LConn1 -- Simulink-PS Converter1/RConn1
  Orifices Tilt/LConn1 -- Simulink-PS Converter/RConn1
  Orifices Lift/LConn3 -- CV LiftB/LConn1 -- PRV LiftA/RConn1 -- CV TiltA/LConn1 -- PRV TiltA/RConn1 -- Orifices Tilt/LConn3 -- PRV Pump/RConn1 -- Orifices Lift/RConn3 -- T/RConn1 -- Orifices Tilt/RConn3 -- CV TiltB/LConn1 -- PRV TiltB/RConn1 -- PRV LiftB/RConn1 -- CV LiftA/LConn1
  CV Lift/LConn1 -- Flow Divider/RConn1
  CV Tilt/LConn1 -- Flow Divider/RConn2
  P/RConn1 -- Flow Divider/LConn1 -- PRV Pump/LConn1

== system sm_wheel_loader_lib/Wheel Loader Vehicle/Actuators/Ideal/Power Draw ==
  pwr : Inport
  Constant : Constant  Value=-5*1e-3*200
  Divide : Product  Inputs=*/
  Gear PTO : sdl_lib/Gears/Simple Gear  ratio=2  rotation_direction=sdl.enum.shaftOutputDirection.opposite  friction_model=sdl.enum.gear_efficiencies_load.off  T_noload=0.1 N*m  T_nom=5 N*m  efficiency_nom=0.8  efficiency=0.8  temperature_TLU=[280, 300, 320] K  load_TLU=[1, 5, 10] N*m  efficiency_TLU=[.95, .9, .85]  efficiency_TLU2=[.85, .8, .75; .95, .9, .85; .85, .8, .7]  w_thr=0.01 rad/s  pwr_thr=0.001 W  enable_backlash=false  hardstop_model=simscape.enum.hardstop.smooth  backlash_distance=1e-3 mm  r_base=0.1 m  transition=1e-4 mm  backlash_stiffness=1e6 N/m  backlash_damping=1e3 N*s/m  coeff_rest=0.7  v_tol=0.001 m/s  f_tol=0.001 N  mu_visc=[0, 0] N*m*s/rad  thermal_mass=50 J/K  temperature_specify=off  temperature_priority=High  temperature=300 K  temperature_nominal_specify=off  temperature_nominal_value=1  temperature_nominal_unit=K  x_backlash_specify=off  x_backlash_priority=None  x_backlash=0 mm  x_backlash_nominal_specify=off  x_backlash_nominal_value=1  x_backlash_nominal_unit=mm  f_hardstop_specify=off  f_hardstop_priority=None  f_hardstop=0 N  f_hardstop_nominal_specify=off  f_hardstop_nominal_value=1  f_hardstop_nominal_unit=N  v_backlash_specify=off  v_backlash_priority=None  v_backlash=0 m/s  v_backlash_nominal_specify=off  v_backlash_nominal_value=1  v_backlash_nominal_unit=m/s
  Ideal Torque Source : fl_lib/Mechanical/Mechanical Sources/Ideal Torque Source
  Limit w : Subsystem
  MRRef : fl_lib/Mechanical/Rotational Elements/Mechanical Rotational Reference
  Motion Sensor : fl_lib/Mechanical/Mechanical Sensors/Ideal Rotational Motion Sensor  reference=foundation.enum.MeasurementReference.difference  acceleration_port=false  velocity_port=true  position_port=true  wrap_angle=false  offset=0 rad
  PS-Simulink Converter : nesl_utility/PS-Simulink Converter  PhysicalDomain=network_engine_domain  SubClassName=ps_output  LeftPortType=input  RightPortType=output  PseudoPeriodic=off  Frequencies=[]  VectorFormat=inherit  Unit=inherit  AffineConversion=off
  Product : Product
  Simulink-PS Converter : nesl_utility/Simulink-PS Converter  PhysicalDomain=network_engine_domain  SubClassName=ps_input  LeftPortType=input  RightPortType=output  PseudoPeriodic=off  Frequencies=[]  NoiseDistribution=none  NoiseParameters=[]  Unit=N*m  AffineConversion=off  FilteringAndDerivatives=provide  SimscapeFilterOrder=1  InputFilterTimeConstant=0.001  UdotUserProvided=0
  Transfer Fcn : TransferFcn  Denominator=[0.01 1]
  PTO : PMIOPort  Side=Right
  wires:
  Product/1 -> Simulink-PS Converter/1
  Transfer Fcn/1 -> Product/2
  PS-Simulink Converter/1 -> Divide/2
  Divide/1 -> Transfer Fcn/1
  pwr/1 -> Divide/1
  Constant/1 -> Product/1
  connections:
  Motion Sensor/RConn2 -- Limit w/LConn1
  Gear PTO/LConn1 -- PTO/RConn1
  MRRef/LConn1 -- Ideal Torque Source/RConn2 -- Motion Sensor/RConn1
  Limit w/RConn1 -- PS-Simulink Converter/LConn1
  Ideal Torque Source/LConn1 -- Motion Sensor/LConn1 -- Gear PTO/RConn1
  Simulink-PS Converter/RConn1 -- Ideal Torque Source/RConn1

== system sm_wheel_loader_lib/Wheel Loader Vehicle/Driveline/Driveline/Driveline 1D ==
  Driveline : Subsystem
      mask Display: image('sm_wheel_loader_driveline1D_IMAGE.png')
  Planetary FL : Subsystem  mask{casing_opc=HMPST.Vis.WhlPlaHou.opc}
      mask prompts: casing_opc "Casing Opacity (0-1)"
      mask Display: image('sm_wheel_loader_driveline_planetaryHubL_IMAGE.png');
  Planetary FR : Subsystem  mask{casing_opc=HMPST.Vis.WhlPlaHou.opc}
      mask prompts: casing_opc "Casing Opacity (0-1)"
      mask Display: image('sm_wheel_loader_driveline_planetaryHubR_IMAGE.png');
  Planetary RL : Subsystem  mask{casing_opc=HMPST.Vis.WhlPlaHou.opc}
      mask prompts: casing_opc "Casing Opacity (0-1)"
      mask Display: image('sm_wheel_loader_driveline_planetaryHubL_IMAGE.png');
  Planetary RR : Subsystem  mask{casing_opc=HMPST.Vis.WhlPlaHou.opc}
      mask prompts: casing_opc "Casing Opacity (0-1)"
      mask Display: image('sm_wheel_loader_driveline_planetaryHubR_IMAGE.png');
  Reference Frame : sm_lib/Frames and Transforms/Reference Frame
  Reference Frame1 : sm_lib/Frames and Transforms/Reference Frame
  wRL : PMIOPort  Side=Left
  Tr1 : PMIOPort  Port=2  Side=Left
  wFL : PMIOPort  Port=3  Side=Left
  HRL : PMIOPort  Port=4  Side=Left
  HRP : PMIOPort  Port=5  Side=Left
  HRR : PMIOPort  Port=6  Side=Left
  wRR : PMIOPort  Port=7  Side=Right
  Tr : PMIOPort  Port=8  Side=Right
  wFR : PMIOPort  Port=9  Side=Right
  HFL : PMIOPort  Port=10  Side=Right
  HFP : PMIOPort  Port=11  Side=Right
  HFR : PMIOPort  Port=12  Side=Right
  connections:
  Tr/RConn1 -- Driveline/RConn2
  Driveline/RConn1 -- Planetary RR/LConn2
  Driveline/RConn3 -- Planetary FR/LConn2
  Driveline/LConn1 -- Planetary RL/RConn2
  Driveline/LConn3 -- Planetary FL/RConn2
  Planetary FR/LConn3 -- HFR/RConn1
  wFR/RConn1 -- Planetary FR/RConn1
  Planetary FL/LConn1 -- wFL/RConn1
  Planetary FL/RConn3 -- HFL/RConn1
  Planetary RR/LConn1 -- HRR/RConn1
  HRL/RConn1 -- Planetary RL/RConn1
  Planetary RL/LConn1 -- wRL/RConn1
  Planetary RR/RConn1 -- wRR/RConn1
  Tr1/RConn1 -- Driveline/LConn2
  HFP/RConn1 -- Reference Frame/RConn1
  Reference Frame1/RConn1 -- HRP/RConn1
